simulink model "ccm_boost_pfc"  (R2021b)
settings: Solver=ode23tb  StartTime=0.0  StopTime=p.duration  MaxStep=p.max_step  RelTol=p.rel_tol  AbsTol=p.abs_tol
values from neighbouring files (symbols this model uses):
  config = [10 1514 1000]    [validate_m1.m]
  event_file = fullfile(folder,[name '_events.csv'])    [event_case.m]    (also in pfc_case.m)
  p = pfc_parameters();p.duration=0.08;p.load_step_time=1    [probe_closed_loop.m]    (also in validate_analog.m = pfc_parameters();p.duration=40e-6;p.max_step=2e-6; validate_control_reset.m = pfc_parameters())
settings Model: Creator=yangs  LastModifiedBy=yangs
settings SolverCC: ZeroCrossControl=EnableAll  ZeroCrossAlgorithm=Adaptive

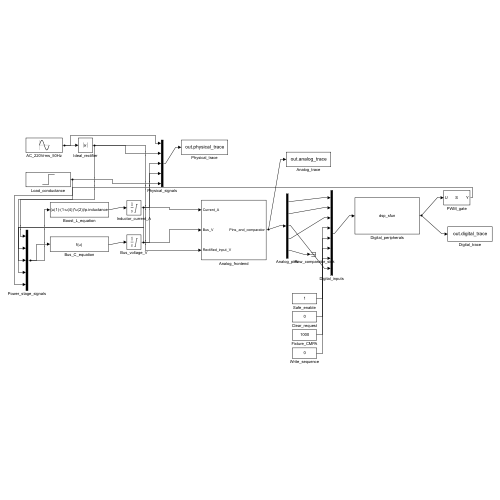
[thumbnail: Simulink's stored preview of the top-level diagram]
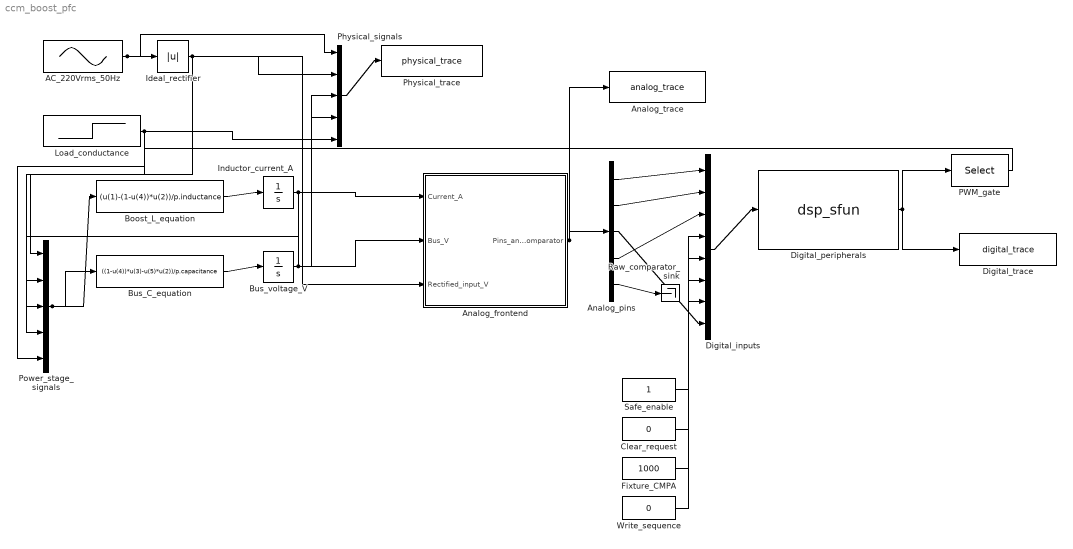
== system ccm_boost_pfc ==
  AC_220Vrms_50Hz : Sin  Amplitude=p.vrms*sqrt(2)  Frequency=2*pi*p.line_hz  SampleTime=0
  Analog_frontend : Subsystem
  Analog_pins : Demux  Outputs=5
  Analog_trace : ToWorkspace  VariableName=analog_trace  SaveFormat=Structure With Time  SampleTime=-1
  Boost_L_equation : Fcn  Expr=(u(1)-(1-u(4))*u(2))/p.inductance
  Bus_C_equation : Fcn  Expr=((1-u(4))*u(3)-u(5)*u(2))/p.capacitance
  Bus_voltage_V : Integrator  InitialCondition=p.initial_vbus  LimitOutput=on  LowerSaturationLimit=0
  Clear_request : Constant  Value=0
  Digital_inputs : Mux  Inputs=8
  Digital_peripherals : S-Function  FunctionName=dsp_sfun  Parameters=config,event_file  SFunctionDeploymentMode=off  EnableBusSupport=off
  Digital_trace : ToWorkspace  VariableName=digital_trace  SaveFormat=Structure With Time  SampleTime=-1
  Fixture_CMPA : Constant  Value=1000
  Ideal_rectifier : Abs
  Inductor_current_A : Integrator  LimitOutput=on  LowerSaturationLimit=0
  Load_conductance : Step  Time=p.load_step_time  Before=p.power_w/p.target_vbus^2  After=p.load_after_w/p.target_vbus^2  SampleTime=0
  PWM_gate : Selector  InputPortWidth=22  IndexOptions=Index vector (dialog)  Indices=1  OutputSizes=1
  Physical_signals : Mux  Inputs=5
  Physical_trace : ToWorkspace  VariableName=physical_trace  SaveFormat=Structure With Time  SampleTime=-1
  Power_stage_signals : Mux  Inputs=5
  Raw_comparator_sink : Terminator
  Safe_enable : Constant
  Write_sequence : Constant  Value=0
  wires:
  AC_220Vrms_50Hz/1 -> Ideal_rectifier/1, Physical_signals/1
  Ideal_rectifier/1 -> Power_stage_signals/1, Analog_frontend/3(Rectified_input_V), Physical_signals/2
  Bus_voltage_V/1 -> Power_stage_signals/2, Analog_frontend/2(Bus_V), Physical_signals/4
  Inductor_current_A/1 -> Power_stage_signals/3, Analog_frontend/1(Current_A), Physical_signals/3
  Load_conductance/1 -> Power_stage_signals/5, Physical_signals/5
  Power_stage_signals/1 -> Boost_L_equation/1, Bus_C_equation/1
  Boost_L_equation/1 -> Inductor_current_A/1
  Bus_C_equation/1 -> Bus_voltage_V/1
  Analog_frontend/1(Pins_and_comparator) -> Analog_pins/1, Analog_trace/1
  Analog_pins/1 -> Digital_inputs/1
  Analog_pins/2 -> Digital_inputs/2
  Analog_pins/4 -> Digital_inputs/3
  Analog_pins/3 -> Digital_inputs/8
  Safe_enable/1 -> Digital_inputs/4
  Clear_request/1 -> Digital_inputs/5
  Fixture_CMPA/1 -> Digital_inputs/6
  Write_sequence/1 -> Digital_inputs/7
  Analog_pins/5 -> Raw_comparator_sink/1
  Digital_inputs/1 -> Digital_peripherals/1
  Digital_peripherals/1 -> Digital_trace/1, PWM_gate/1
  PWM_gate/1 -> Power_stage_signals/4
  Physical_signals/1 -> Physical_trace/1

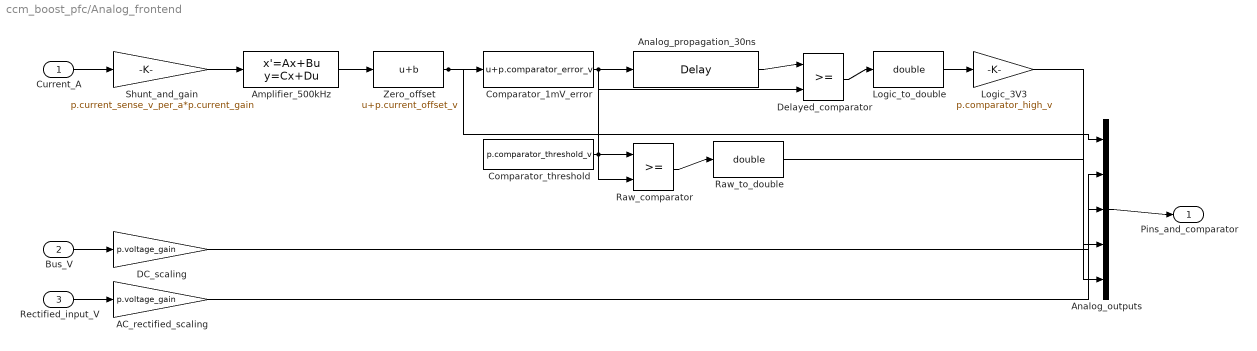
== system ccm_boost_pfc/Analog_frontend ==
  Current_A : Inport
  Bus_V : Inport  Port=2
  Rectified_input_V : Inport  Port=3
  AC_rectified_scaling : Gain  Gain=p.voltage_gain
  Amplifier_500kHz : StateSpace  A=-1/p.current_tau  B=1/p.current_tau  D=0  InitialCondition=0
  Analog_outputs : Mux  Inputs=5
  Analog_propagation_30ns : TransportDelay  DelayTime=p.comparator_delay_s
  Comparator_1mV_error : Bias  Bias=p.comparator_error_v
  Comparator_threshold : Constant  Value=p.comparator_threshold_v
  DC_scaling : Gain  Gain=p.voltage_gain
  Delayed_comparator : RelationalOperator  OutDataTypeStr=boolean  RndMeth=Simplest
  Logic_3V3 : Gain  Gain=p.comparator_high_v
  Logic_to_double : DataTypeConversion  OutDataTypeStr=double
  Raw_comparator : RelationalOperator  OutDataTypeStr=boolean  RndMeth=Simplest
  Raw_to_double : DataTypeConversion  OutDataTypeStr=double
  Shunt_and_gain : Gain  Gain=p.current_sense_v_per_a*p.current_gain
  Zero_offset : Bias  Bias=p.current_offset_v
  Pins_and_comparator : Outport
  wires:
  Current_A/1 -> Shunt_and_gain/1
  Shunt_and_gain/1 -> Amplifier_500kHz/1
  Amplifier_500kHz/1 -> Zero_offset/1
  Bus_V/1 -> DC_scaling/1
  Rectified_input_V/1 -> AC_rectified_scaling/1
  Zero_offset/1 -> Comparator_1mV_error/1, Analog_outputs/1
  Comparator_1mV_error/1 -> Analog_propagation_30ns/1, Raw_comparator/1
  Analog_propagation_30ns/1 -> Delayed_comparator/1
  Comparator_threshold/1 -> Delayed_comparator/2, Raw_comparator/2
  Delayed_comparator/1 -> Logic_to_double/1
  Logic_to_double/1 -> Logic_3V3/1
  Raw_comparator/1 -> Raw_to_double/1
  DC_scaling/1 -> Analog_outputs/2
  AC_rectified_scaling/1 -> Analog_outputs/3
  Logic_3V3/1 -> Analog_outputs/4
  Raw_to_double/1 -> Analog_outputs/5
  Analog_outputs/1 -> Pins_and_comparator/1
